simulink model "DC_Motorr"  (R2023b)
settings: Solver=FixedStepAuto  StartTime=0.0  StopTime=2000  FixedStep=1e-3  RelTol=1e-3
values from neighbouring files (symbols this model uses):
  beta = 0.81    [DC_Motor.m]
  d = 0.68    [DC_Motor.m]
  En = 600 - Ra*156    (= 539.16)    [DC_Motor.m]
  I_en = 5    [DC_Motor.m]
  Ia_max = 156    [DC_Motor.m]
  Jeq = m_total * (rho^2 * d^2) / 4    (= 90.6180715851)    [DC_Motor.m]
  Ki_ia = C_a.Ki    [DC_Motor.m]
  Ki_ie = C_e.Ki    [DC_Motor.m]
  Ki_v = C_M.Ki    [DC_Motor.m]
  Kp_ia = C_a.Kp    [DC_Motor.m]
  Kp_ie = C_e.Kp    [DC_Motor.m]
  Kp_v = C_M.Kp    [DC_Motor.m]
  Kt = 1.06    [DC_Motor.m]
  L = [0,1,3,4,6,8,9,10]    [DC_Motor.m]
  La = tau_a * Ra    (= 0.0039)    [DC_Motor.m]
  Le = tau_e * Re    (= 1.2)    [DC_Motor.m]
  m_total = m_tram + m_passengers    (= 25400)    [DC_Motor.m]
  Omega_b = 970 * (2*pi/60)    (= 101.578162466)    [DC_Motor.m]
  Ra = 0.39    [DC_Motor.m]
  Re = 12    [DC_Motor.m]
  rho = 13/74    (= 0.175675675676)    [DC_Motor.m]
  S_ref = [0, 0, 5, 0, 0, -5, 0, 0] / 100    [DC_Motor.m]
  tau_a = 10e-3    (= 0.01)    [DC_Motor.m]
  V_max = 42 * (1000/3600)    (= 11.6666666667)    [DC_Motor.m]
  V_ref = [V_r/2,V_r,V_r,V_max,V_r,V_r,V_r/2,0]    [DC_Motor.m]
libraries: slpidlib x3
settings Model: Creator=ASUS  LastModifiedBy=HP Elite
settings RTWCC: GPUComputeCapability=5.0

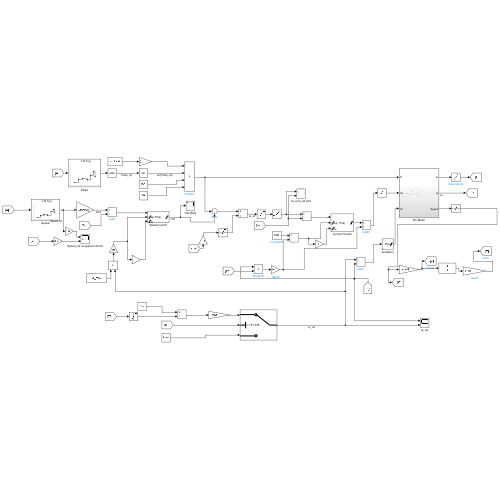
[thumbnail: Simulink's stored preview of the top-level diagram]
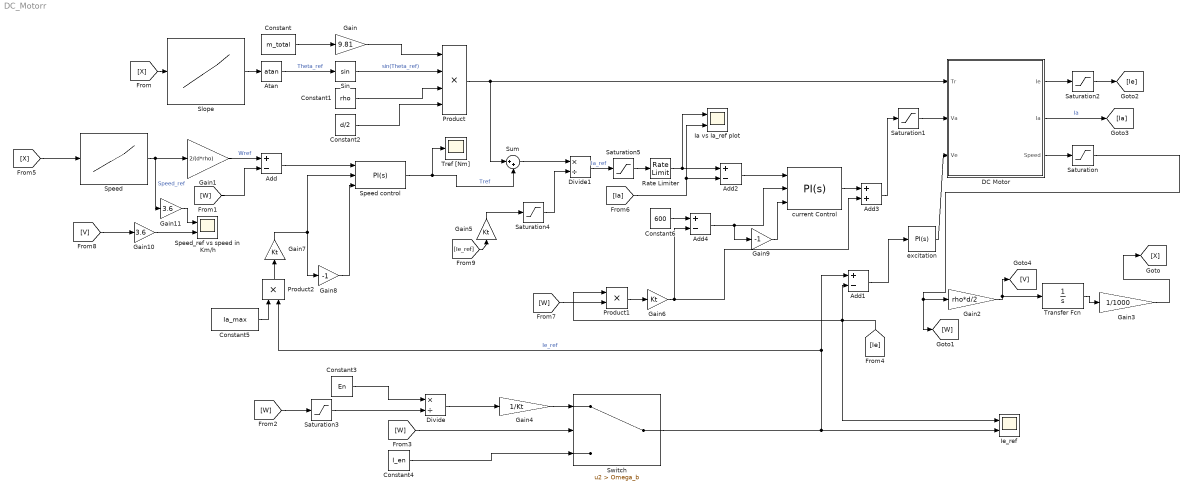
== system DC_Motorr ==
  Add{,1..2,4} (4 alike) : Sum  Inputs=+-
  Add3 : Sum
  Atan : Trigonometry  Operator=atan
  Constant : Constant  Value=m_total
  Constant1 : Constant  Value=rho
  Constant2 : Constant  Value=d/2
  Constant3 : Constant  Value=En
  Constant4 : Constant  Value=I_en
  Constant5 : Constant  Value=Ia_max
  Constant6 : Constant  Value=600
  DC Motor : Subsystem
  Divide : Product  Inputs=*/
  Divide1 : Product  Inputs=*/
  Gain : Gain  Gain=9.81
  Gain1 : Gain  Gain=2/(d*rho)
  Gain10 : Gain  Gain=3.6
  Gain11 : Gain  Gain=3.6
  Gain2 : Gain  Gain=rho*d/2
  Gain3 : Gain  Gain=1/1000
  Gain4 : Gain  Gain=1/Kt
  Gain5 : Gain  Gain=Kt
  Gain6 : Gain  Gain=Kt
  Gain7 : Gain  Gain=Kt
  Gain8 : Gain  Gain=-1
  Gain9 : Gain  Gain=-1
  Ia vs Ia_ref plot : Scope  NumInputPorts=2
  Ie_ref : Scope  NumInputPorts=2
  Product : Product  Inputs=4
  Product1 : Product
  Product2 : Product
  Rate Limiter : RateLimiter  RisingSlewLimit=Ia_max/tau_a  FallingSlewLimit=-Ia_max/tau_a  SampleTimeMode=inherited
  Saturation : Saturate  UpperLimit=V_max/ (rho*d/2)  LowerLimit=-V_max/ (rho*d/2)
  Saturation1 : Saturate  UpperLimit=600  LowerLimit=-600
  Saturation2 : Saturate  UpperLimit=5  LowerLimit=0.00001
  Saturation3 : Saturate  UpperLimit=inf  LowerLimit=Omega_b
  Saturation4 : Saturate  UpperLimit=inf  LowerLimit=2
  Saturation5 : Saturate  UpperLimit=156  LowerLimit=-156
  Sin : Trigonometry
  Slope : Lookup_n-D  NumberOfTableDimensions=1  LookupTableObject=''  BreakpointsForDimension1=L  BreakpointsForDimension2=[1:2]  BreakpointsForDimension3=[5, 7]  BreakpointsForDimension1FirstPoint=10  BreakpointsForDimension2FirstPoint=10  BreakpointsForDimension1Spacing=12  BreakpointsForDimension2Spacing=12  Table=S_ref  InterpMethod=Flat  DiagnosticForOutOfRangeInput=Warning  InternalRulePriority=Speed  RndMeth=Simplest
  Speed : Lookup_n-D  NumberOfTableDimensions=1  BreakpointsForDimension1=L  Table=V_ref  InterpMethod=Flat  InternalRulePriority=Speed  RndMeth=Simplest
  Speed control : slpidlib/PID Controller  Controller=PI  Form=Parallel  TimeDomain=Continuous-time  UseExternalTs=off  SampleTime=-1  IntegratorMethod=Forward Euler  FilterMethod=Forward Euler  ControllerParametersSource=internal  P=Kp_v  I=Ki_v  UseKiTs=off  D=0  N=100  UseFilter=on  TunerSelectOption=Transfer Function Based (PID Tuner App)  InitialConditionSource=internal  InitialConditionForIntegrator=0  InitialConditionForFilter=0  DifferentiatorICPrevScaledInput=0  ExternalReset=none  TrackingMode=off  Kt=1  LimitOutput=on  SatLimitsSource=external  UpperSaturationLimit=826.8  LowerSaturationLimit=-826.8  LinearizeAsGain=on  AntiWindupMode=back-calculation  Kb=Ki_v/Kp_v  LimitIntegrator=on  UpperIntegratorSaturationLimit=826.8  LowerIntegratorSaturationLimit=-826.8  RndMeth=Nearest  POutMin=[]  POutMax=[]  IOutMin=[]  IOutMax=[]  DOutMin=[]  DOutMax=[]  NOutMin=[]  NOutMax=[]  SumOutMin=[]  SumOutMax=[]  SaturationOutMin=[]  SaturationOutMax=[]  PParamMin=[]  PParamMax=[]  IParamMin=[]  IParamMax=[]  DParamMin=[]  DParamMax=[]  NParamMin=[]  NParamMax=[]  KbParamMin=[]  KbParamMax=[]  KtParamMin=[]  KtParamMax=[]  KbOutMin=[]  KbOutMax=[]  KtOutMin=[]  KtOutMax=[]  IntegratorOutMin=[]  IntegratorOutMax=[]  FilterOutMin=[]  FilterOutMax=[]  SumI1OutMin=[]  SumI1OutMax=[]  SumI2OutMin=[]  SumI2OutMax=[]  SumI3OutMin=[]  SumI3OutMax=[]  SumI4OutMin=[]  SumI4OutMax=[]  SumDOutMin=[]  SumDOutMax=[]  DifferentiatorOutMin=[]  DifferentiatorOutMax=[]  FilterDiffOutCoefMin=[]  FilterDiffOutCoefMax=[]  ReciprocalOutMin=[]  ReciprocalOutMax=[]  SumDenOutMin=[]  SumDenOutMax=[]  SumNumOutMin=[]  SumNumOutMax=[]  DivideOutMin=[]  DivideOutMax=[]  UdiffTsProdOutMin=[]  UdiffTsProdOutMax=[]  NTsProdOutMin=[]  NTsProdOutMax=[]  UintegralTsProdOutMin=[]  UintegralTsProdOutMax=[]  UngainTsProdOutMin=[]  UngainTsProdOutMax=[]  ClampingZeroOutDataTypeStr=Inherit: Inherit via back propagation  ClampingZeroOutMin=[]  ClampingZeroOutMax=[]  FilterDenConstantOutDataTypeStr=Inherit: Inherit via back propagation  FilterDenConstantOutMin=[]  FilterDenConstantOutMax=[]  PCopyOutDataTypeStr=Inherit: Inherit via back propagation  PCopyOutMin=[]  PCopyOutMax=[]  NCopyOutDataTypeStr=Inherit: Inherit via back propagation  NCopyOutMin=[]  NCopyOutMax=[]  IntegratorContinuousStateAttributes=''  IntegratorStateMustResolveToSignalObject=off  IntegratorRTWStateStorageClass=Auto  FilterContinuousStateAttributes=''  FilterStateMustResolveToSignalObject=off  FilterRTWStateStorageClass=Auto  ParallelPVariant=InternalParameters  IdealPVariant=Disabled  IVariant=InternalParameters  DVariant=Disabled  IntegratorVariant=Continuous  SatVariant=External  AWVariant=BackCalculation  PCopyVariant=Disabled  TRVariant=Disabled  FdbkBlocksVariant=Forward  IdealPFdbkVariant=Disabled  SatFdbkVariant=Disabled  DerivativeFilterVariant=Disabled  NVariant=Disabled  NCopyVariant=Disabled_SignalSpec  FilterICVariant=Disabled  IntegratorICVariant=InternalICs  ExternalResetVariant=Disabled  TRSumVariant=Passthrough  SumFdbkVariant=Disabled  SumVariant=Sum_PI  TsampFilterVariant=InternalTs  TsampNgainVariant=Passthrough  TsampIntegralVariant=Disabled_SignalSpec  ExternalSaturationOutDataTypeStr=Inherit: Same as second input
  Speed_ref vs speed in Km/h : Scope  NumInputPorts=2
  Sum : Sum  Inputs=|++
  Switch : Switch  Criteria=u2 > Threshold  Threshold=Omega_b  SaturateOnIntegerOverflow=off  InputSameDT=off
  Transfer Fcn : TransferFcn  Denominator=[1 0]
  Tref [Nm] : Scope
  current Control : slpidlib/PID Controller  Controller=PI  Form=Parallel  TimeDomain=Continuous-time  UseExternalTs=off  SampleTime=-1  IntegratorMethod=Forward Euler  FilterMethod=Forward Euler  ControllerParametersSource=internal  P=Kp_ia  I=Ki_ia  UseKiTs=off  D=0  N=100  UseFilter=on  TunerSelectOption=Transfer Function Based (PID Tuner App)  InitialConditionSource=internal  InitialConditionForIntegrator=0  InitialConditionForFilter=0  DifferentiatorICPrevScaledInput=0  ExternalReset=none  TrackingMode=off  Kt=1  LimitOutput=on  SatLimitsSource=external  UpperSaturationLimit=600  LowerSaturationLimit=-600  LinearizeAsGain=off  AntiWindupMode=back-calculation  Kb=Ki_ia/Kp_ia  LimitIntegrator=off  UpperIntegratorSaturationLimit=600  LowerIntegratorSaturationLimit=-600  POutMin=[]  POutMax=[]  IOutMin=[]  IOutMax=[]  DOutMin=[]  DOutMax=[]  NOutMin=[]  NOutMax=[]  SumOutMin=[]  SumOutMax=[]  SaturationOutMin=[]  SaturationOutMax=[]  PParamMin=[]  PParamMax=[]  IParamMin=[]  IParamMax=[]  DParamMin=[]  DParamMax=[]  NParamMin=[]  NParamMax=[]  KbParamMin=[]  KbParamMax=[]  KtParamMin=[]  KtParamMax=[]  KbOutMin=[]  KbOutMax=[]  KtOutMin=[]  KtOutMax=[]  IntegratorOutMin=[]  IntegratorOutMax=[]  FilterOutMin=[]  FilterOutMax=[]  SumI1OutMin=[]  SumI1OutMax=[]  SumI2OutMin=[]  SumI2OutMax=[]  SumI3OutMin=[]  SumI3OutMax=[]  SumI4OutMin=[]  SumI4OutMax=[]  SumDOutMin=[]  SumDOutMax=[]  DifferentiatorOutMin=[]  DifferentiatorOutMax=[]  FilterDiffOutCoefMin=[]  FilterDiffOutCoefMax=[]  ReciprocalOutMin=[]  ReciprocalOutMax=[]  SumDenOutMin=[]  SumDenOutMax=[]  SumNumOutMin=[]  SumNumOutMax=[]  DivideOutMin=[]  DivideOutMax=[]  UdiffTsProdOutMin=[]  UdiffTsProdOutMax=[]  NTsProdOutMin=[]  NTsProdOutMax=[]  UintegralTsProdOutMin=[]  UintegralTsProdOutMax=[]  UngainTsProdOutMin=[]  UngainTsProdOutMax=[]  ClampingZeroOutDataTypeStr=Inherit: Inherit via back propagation  ClampingZeroOutMin=[]  ClampingZeroOutMax=[]  FilterDenConstantOutDataTypeStr=Inherit: Inherit via back propagation  FilterDenConstantOutMin=[]  FilterDenConstantOutMax=[]  PCopyOutDataTypeStr=Inherit: Inherit via back propagation  PCopyOutMin=[]  PCopyOutMax=[]  NCopyOutDataTypeStr=Inherit: Inherit via back propagation  NCopyOutMin=[]  NCopyOutMax=[]  IntegratorContinuousStateAttributes=''  IntegratorStateMustResolveToSignalObject=off  IntegratorRTWStateStorageClass=Auto  FilterContinuousStateAttributes=''  FilterStateMustResolveToSignalObject=off  FilterRTWStateStorageClass=Auto  ParallelPVariant=InternalParameters  IdealPVariant=Disabled  IVariant=InternalParameters  DVariant=Disabled  IntegratorVariant=Continuous  SatVariant=External  AWVariant=BackCalculation  PCopyVariant=Disabled  TRVariant=Disabled  FdbkBlocksVariant=Forward  IdealPFdbkVariant=Disabled  SatFdbkVariant=Disabled  DerivativeFilterVariant=Disabled  NVariant=Disabled  NCopyVariant=Disabled_SignalSpec  FilterICVariant=Disabled  IntegratorICVariant=InternalICs  ExternalResetVariant=Disabled  TRSumVariant=Passthrough  SumFdbkVariant=Disabled  SumVariant=Sum_PI  TsampFilterVariant=InternalTs  TsampNgainVariant=Passthrough  TsampIntegralVariant=Disabled_SignalSpec  ExternalSaturationOutDataTypeStr=Inherit: Same as second input
  excitation : slpidlib/PID Controller  Controller=PI  Form=Parallel  TimeDomain=Continuous-time  UseExternalTs=off  SampleTime=-1  IntegratorMethod=Forward Euler  FilterMethod=Forward Euler  ControllerParametersSource=internal  P=Kp_ie  I=Ki_ie  UseKiTs=off  D=0  N=100  UseFilter=on  TunerSelectOption=Transfer Function Based (PID Tuner App)  InitialConditionSource=internal  InitialConditionForIntegrator=0  InitialConditionForFilter=0  DifferentiatorICPrevScaledInput=0  ExternalReset=none  TrackingMode=off  Kt=1  LimitOutput=on  SatLimitsSource=internal  UpperSaturationLimit=60  LowerSaturationLimit=-60  LinearizeAsGain=on  AntiWindupMode=back-calculation  Kb=Ki_ie/Kp_ie  LimitIntegrator=off  UpperIntegratorSaturationLimit=60  LowerIntegratorSaturationLimit=-60  POutMin=[]  POutMax=[]  IOutMin=[]  IOutMax=[]  DOutMin=[]  DOutMax=[]  NOutMin=[]  NOutMax=[]  SumOutMin=[]  SumOutMax=[]  SaturationOutMin=[]  SaturationOutMax=[]  PParamMin=[]  PParamMax=[]  IParamMin=[]  IParamMax=[]  DParamMin=[]  DParamMax=[]  NParamMin=[]  NParamMax=[]  KbParamMin=[]  KbParamMax=[]  KtParamMin=[]  KtParamMax=[]  KbOutMin=[]  KbOutMax=[]  KtOutMin=[]  KtOutMax=[]  IntegratorOutMin=[]  IntegratorOutMax=[]  FilterOutMin=[]  FilterOutMax=[]  SumI1OutMin=[]  SumI1OutMax=[]  SumI2OutMin=[]  SumI2OutMax=[]  SumI3OutMin=[]  SumI3OutMax=[]  SumI4OutMin=[]  SumI4OutMax=[]  SumDOutMin=[]  SumDOutMax=[]  DifferentiatorOutMin=[]  DifferentiatorOutMax=[]  FilterDiffOutCoefMin=[]  FilterDiffOutCoefMax=[]  ReciprocalOutMin=[]  ReciprocalOutMax=[]  SumDenOutMin=[]  SumDenOutMax=[]  SumNumOutMin=[]  SumNumOutMax=[]  DivideOutMin=[]  DivideOutMax=[]  UdiffTsProdOutMin=[]  UdiffTsProdOutMax=[]  NTsProdOutMin=[]  NTsProdOutMax=[]  UintegralTsProdOutMin=[]  UintegralTsProdOutMax=[]  UngainTsProdOutMin=[]  UngainTsProdOutMax=[]  ClampingZeroOutDataTypeStr=Inherit: Inherit via back propagation  ClampingZeroOutMin=[]  ClampingZeroOutMax=[]  FilterDenConstantOutDataTypeStr=Inherit: Inherit via back propagation  FilterDenConstantOutMin=[]  FilterDenConstantOutMax=[]  PCopyOutDataTypeStr=Inherit: Inherit via back propagation  PCopyOutMin=[]  PCopyOutMax=[]  NCopyOutDataTypeStr=Inherit: Inherit via back propagation  NCopyOutMin=[]  NCopyOutMax=[]  IntegratorContinuousStateAttributes=''  IntegratorStateMustResolveToSignalObject=off  IntegratorRTWStateStorageClass=Auto  FilterContinuousStateAttributes=''  FilterStateMustResolveToSignalObject=off  FilterRTWStateStorageClass=Auto  ParallelPVariant=InternalParameters  IdealPVariant=Disabled  IVariant=InternalParameters  DVariant=Disabled  IntegratorVariant=Continuous  SatVariant=Enabled  AWVariant=BackCalculation  PCopyVariant=Disabled  TRVariant=Disabled  FdbkBlocksVariant=Forward  IdealPFdbkVariant=Disabled  SatFdbkVariant=Disabled  DerivativeFilterVariant=Disabled  NVariant=Disabled  NCopyVariant=Disabled_SignalSpec  FilterICVariant=Disabled  IntegratorICVariant=InternalICs  ExternalResetVariant=Disabled  TRSumVariant=Passthrough  SumFdbkVariant=Disabled  SumVariant=Sum_PI  TsampFilterVariant=InternalTs  TsampNgainVariant=Passthrough  TsampIntegralVariant=Disabled_SignalSpec  ExternalSaturationOutDataTypeStr=Inherit: Same as second input
  wires:
  Slope/1 -> Atan/1
  Atan/1 -> Sin/1  "Theta_ref"
  Constant/1 -> Gain/1
  Gain/1 -> Product/1
  Sin/1 -> Product/2  "sin(Theta_ref)"
  Constant1/1 -> Product/3
  Constant2/1 -> Product/4
  Speed/1 -> Gain11/1, Gain1/1  "Speed_ref"
  Gain1/1 -> Add/1  "Wref"
  DC Motor/3(Speed) -> Saturation/1
  Saturation/1 -> [W], Gain2/1
  Gain2/1 -> [V], Transfer Fcn/1
  Transfer Fcn/1 -> Gain3/1
  Gain3/1 -> [X]
  [X] -> Slope/1
  [W] -> Add/2
  Constant3/1 -> Divide/1
  [W] -> Switch/2
  Constant4/1 -> Switch/3
  Divide/1 -> Gain4/1
  Gain4/1 -> Switch/1
  Switch/1 -> Add1/1, Product2/2, Ie_ref/2  "Ie_ref"
  [Ie] -> Product1/1, Add1/2, Ie_ref/1
  Add1/1 -> excitation/1
  excitation/1 -> DC Motor/3(Ve)
  [X] -> Speed/1
  Add/1 -> Speed control/1
  [Ia] -> Ia vs Ia_ref plot/2, Add2/2
  Gain6/1 -> Add3/2, Add4/2
  Product1/1 -> Gain6/1
  [W] -> Product1/2
  Add3/1 -> Saturation1/1
  Product2/1 -> Gain7/1
  Constant5/1 -> Product2/1
  Gain7/1 -> Speed control/2, Gain8/1
  Speed control/1 -> Sum/2, Tref [Nm]/1  "Tref"
  DC Motor/1(Ie) -> Saturation2/1
  Constant6/1 -> Add4/1
  Product/1 -> Sum/1, DC Motor/1(Tr)
  Gain8/1 -> Speed control/3
  Saturation2/1 -> [Ie]
  Add4/1 -> current Control/2, Gain9/1
  Add2/1 -> current Control/1
  Saturation1/1 -> DC Motor/2(Va)
  current Control/1 -> Add3/1
  Gain9/1 -> current Control/3
  Saturation3/1 -> Divide/2
  [W] -> Saturation3/1
  Sum/1 -> Divide1/1
  [V] -> Gain10/1
  Gain10/1 -> Speed_ref vs speed in Km/h/2
  Gain11/1 -> Speed_ref vs speed in Km/h/1
  [Ie_ref] -> Gain5/1
  Gain5/1 -> Saturation4/1
  Saturation4/1 -> Divide1/2
  DC Motor/2(Ia) -> [Ia]  "Ia"
  Saturation5/1 -> Rate Limiter/1
  Divide1/1 -> Saturation5/1  "Ia_ref"
  Rate Limiter/1 -> Ia vs Ia_ref plot/1, Add2/1

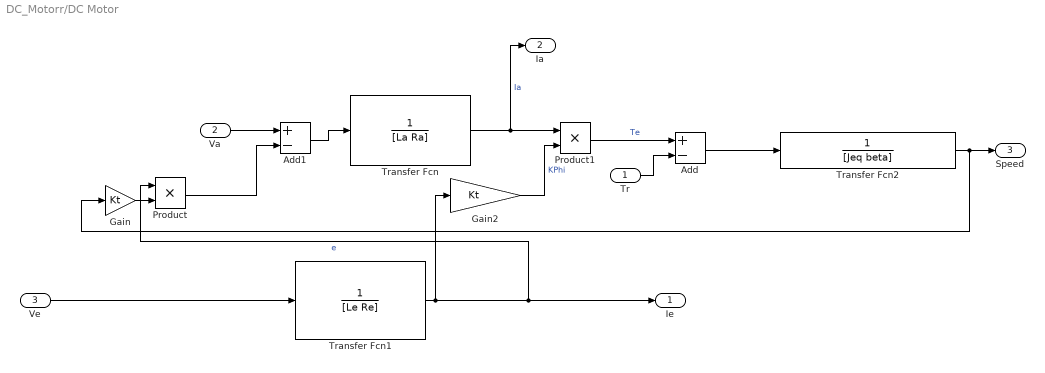
== system DC_Motorr/DC Motor ==
  Tr : Inport
  Va : Inport  Port=2
  Ve : Inport  Port=3
  Add : Sum  Inputs=+-
  Add1 : Sum  Inputs=+-
  Gain : Gain  Gain=Kt
  Gain2 : Gain  Gain=Kt
  Product : Product
  Product1 : Product
  Transfer Fcn : TransferFcn  Denominator=[La Ra]
  Transfer Fcn1 : TransferFcn  Denominator=[Le Re]
  Transfer Fcn2 : TransferFcn  Denominator=[Jeq beta]
  Ie : Outport
  Ia : Outport  Port=2
  Speed : Outport  Port=3
  wires:
  Transfer Fcn1/1 -> Product/1, Ie/1, Gain2/1  "e"
  Ve/1 -> Transfer Fcn1/1
  Transfer Fcn/1 -> Ia/1, Product1/1  "Ia"
  Transfer Fcn2/1 -> Gain/1, Speed/1
  Gain2/1 -> Product1/2  "KPhi"
  Product1/1 -> Add/1  "Te"
  Tr/1 -> Add/2
  Add/1 -> Transfer Fcn2/1
  Va/1 -> Add1/1
  Add1/1 -> Transfer Fcn/1
  Gain/1 -> Product/2
  Product/1 -> Add1/2
